simulink model "pgfm_ctrl_analysis"  (R2026b)
settings: Solver=ode23t  StopTime=param.sim.simlength  FixedStep=param.sim.tc  MaxStep=param.glb_time.tc  RelTol=1e-4
values from neighbouring files (symbols this model uses):
  param = add_template_extras(param, options)    [init_model.m]
undefined symbols (not defined in the file or in its folder): magnitude
libraries: fl_lib x99, nesl_utility x59, afe_uvw_ctrl x15, discrete_time_low_pass_filter x3, threephase_inductor_lib x3, dclink_for_two_levels x3, three_phase_pwm_modulator x3, ideal_bridges_lib x3, lithium_ion_battery x1, three_phase_voltage_with_frt_emulator_mfcn x1
(part 4 of 6)

== system pgfm_ctrl_analysis/afe_abc_inv_psm_mod2/AFE_control/afe_control/FRT-VDE4110 ==
  Constant4 : Constant  Value=0
  Mux : Mux
  Mux1 : Mux  Inputs=2
  enable : Step  Time=param.frt.data.settle_time  FinalValue=param.frt.data.enable_frt_1 + param.frt.data.enable_frt_2
  frt_detection_output : Scope  Commented=on  NumInputPorts=3
      settings: ActiveDisplayYMinimum=-0.12499999999999997  ActiveDisplayYMaximum=1.125
  frt_vde4110 : afe_uvw_ctrl/frt_vde4110  p=param.afe.uvw
  positive_reactive_current_reference : Subsystem
  reset : Step  Time=0.025  InitialValue=1  FinalValue=0
  tag scope: frt_active=scoped, i_grid_seq_ref=scoped, pwr_lim_enable=scoped
  wires:
  Mux1/1 -> frt_vde4110/2
  [i_react_pos_ref] -> Mux1/1
  [i_react_neg_ref] -> Mux1/2
  frt_vde4110/1 -> [i_grid_seq_ref]
  Constant4/1 -> [i_react_neg_ref]
  positive_reactive_current_reference/1(i_react_pos_ref) -> [i_react_pos_ref]
  Mux/1 -> frt_vde4110/1
  [v_grid_pos_xi_avg] -> Mux/1
  [v_grid_pos_eta_avg] -> Mux/2
  [v_grid_neg_xi_avg] -> Mux/3
  [v_grid_neg_eta_avg] -> Mux/4
  enable/1 -> frt_vde4110/3  "enable"
  reset/1 -> frt_vde4110/4  "reset"
  frt_vde4110/4 -> frt_detection_output/1  "frt_state"
  frt_vde4110/3 -> frt_detection_output/3, [pwr_lim_enable]  "pwr_lim_enable"
  frt_vde4110/2 -> frt_detection_output/2, [frt_active]  "frt_active"

== system pgfm_ctrl_analysis/afe_abc_inv_psm_mod2/AFE_control/afe_control/current_ctrl ==
  i_xi_ref : Inport
  Mux : Mux  Inputs=3
  current_ctrl_uvw : afe_uvw_ctrl/current_ctrl_uvw  p=param.afe.uvw
  isa_ref/isa : Scope  Commented=on  NumInputPorts=2
      settings: ActiveDisplayYMinimum=-3.5647345146351177  ActiveDisplayYMaximum=2.2290599372806974
  u_alpha_beta_gamma_out : Outport
  wires:
  Mux/1 -> current_ctrl_uvw/2
  current_ctrl_uvw/3 -> isa_ref/isa/2
  current_ctrl_uvw/2 -> isa_ref/isa/1
  current_ctrl_uvw/1 -> u_alpha_beta_gamma_out/1
  [isd_abc_pu] -> current_ctrl_uvw/3
  [phase_grid_pll] -> current_ctrl_uvw/4
  [i_stack_neg_eta_ref] -> Mux/3  "is_neg_eta_ref"
  [i_stack_pos_eta_ref] -> Mux/1  "is_pos_eta_ref"
  [i_stack_neg_xi_ref] -> Mux/2  "is_neg_xi_ref"
  i_xi_ref/1 -> current_ctrl_uvw/1  "is_pos_xi_ref"

== system pgfm_ctrl_analysis/afe_abc_inv_psm_mod2/AFE_control/afe_control/data_to_worspace_module_1 ==
  Bus Creator : BusCreator  Inputs=5
  dq_pll : Subsystem
  inner_current_tracking : Subsystem
  pwr_meter : Subsystem
  sequences_data : Subsystem
  m : Outport
  wires:
  dq_pll/1(dqPLLs) -> Bus Creator/4  "dq_pll"
  [local_time] -> Bus Creator/5  "local_time"
  inner_current_tracking/1(m_inner_current_tracking) -> Bus Creator/3  "m_inner_current_tracking"
  pwr_meter/1(m_pwr_meter) -> Bus Creator/2  "pwr_meter"
  sequences_data/1(m_seq) -> Bus Creator/1  "sequences_data"
  Bus Creator/1 -> m/1

== system pgfm_ctrl_analysis/afe_abc_inv_psm_mod2/AFE_control/afe_control/grid_current_sequences_and_reactive_pwr_ctrl ==
  ig_abc_pu : Inport
  Abs : Abs  SaturateOnIntegerOverflow=off
  Demux : Demux  Outputs=3
  Demux1 : Demux
  Saturation : Saturate  UpperLimit=2  LowerLimit=0.1
  Terminator : Terminator
  grid_current_sequences_q_ctrl : afe_uvw_ctrl/grid_current_sequences_q_ctrl  p=param.afe.uvw
  tag scope: i_grid_neg_eta_avg=scoped, i_grid_neg_xi_avg=scoped, i_grid_pos_eta_avg=scoped, i_grid_pos_xi_avg=scoped, i_stack_neg_eta_ref=scoped, i_stack_neg_xi_ref=scoped, i_stack_pos_eta_ref=scoped
  wires:
  Demux/3 -> [i_stack_neg_eta_ref]
  Demux/2 -> [i_stack_neg_xi_ref]
  Abs/1 -> Saturation/1
  [omega_grid_pll_pu] -> Abs/1
  Saturation/1 -> grid_current_sequences_q_ctrl/3
  [i_grid_seq_ref] -> grid_current_sequences_q_ctrl/4
  grid_current_sequences_q_ctrl/3 -> Terminator/1
  Demux1/4 -> [i_grid_neg_eta_avg]
  Demux1/3 -> [i_grid_neg_xi_avg]
  Demux1/2 -> [i_grid_pos_eta_avg]
  Demux1/1 -> [i_grid_pos_xi_avg]
  grid_current_sequences_q_ctrl/2 -> Demux1/1
  Demux/1 -> [i_stack_pos_eta_ref]
  grid_current_sequences_q_ctrl/1 -> Demux/1
  ig_abc_pu/1 -> grid_current_sequences_q_ctrl/1
  [phase_grid_pll] -> grid_current_sequences_q_ctrl/2

== system pgfm_ctrl_analysis/afe_abc_inv_psm_mod2/AFE_control/afe_control/grid_phase_acquisition ==
  grid_phase : Inport
  Quantizer : Quantizer  QuantizationInterval=param.meas.adc_quantization
  Unit Delay : UnitDelay  SampleTime=-1
  Zero-Order Hold : ZeroOrderHold  SampleTime=-1
  grid_phased : Outport
  wires:
  Quantizer/1 -> Unit Delay/1
  grid_phase/1 -> Zero-Order Hold/1
  Unit Delay/1 -> grid_phased/1
  Zero-Order Hold/1 -> Quantizer/1

== system pgfm_ctrl_analysis/afe_abc_inv_psm_mod2/AFE_control/afe_control/grid_voltage_phase_lock_loops ==
  ug_abc_pu : Inport
  Bus Creator2 : BusCreator  Inputs=2
  FHT-PLL performance : Scope  Commented=on  NumInputPorts=2
      settings: ActiveDisplayYMinimum=-1.32501220703125  ActiveDisplayYMaximum=1.30987548828125  DataLoggingVariableName=ScopeData8
  FHT-PLL_simulink : Subsystem
  tag scope: omega_grid_pll_pu=scoped, phase_grid_pll=scoped
  wires:
  [phase_grid_pll] -> Bus Creator2/1  "phase_grid_fht_pll"
  [omega_grid_pll_pu] -> Bus Creator2/2  "omega_grid_fht_pll"
  Bus Creator2/1 -> FHT-PLL performance/2
  ug_abc_pu/1 -> FHT-PLL_simulink/1(ug_abc_pu), FHT-PLL performance/1
  FHT-PLL_simulink/2(omega_grid_fht_pll) -> [omega_grid_pll_pu]
  FHT-PLL_simulink/1(gamma_grid_fht_pll) -> [phase_grid_pll]

== system pgfm_ctrl_analysis/afe_abc_inv_psm_mod2/AFE_control/afe_control/grid_voltage_sequences ==
  Abs : Abs  SaturateOnIntegerOverflow=off
  Demux : Demux
  Demux1 : Demux  Outputs=2
  Saturation : Saturate  UpperLimit=2  LowerLimit=0.1
  Terminator : Terminator
  grid_voltage_sequences1 : afe_uvw_ctrl/grid_voltage_sequences  p=param.afe.uvw
  tag scope: ug_alpha_pu=scoped, ug_beta_pu=scoped, v_grid_neg_eta_avg=scoped, v_grid_neg_xi_avg=scoped, v_grid_pos_eta_avg=scoped, v_grid_pos_xi_avg=scoped
  wires:
  grid_voltage_sequences1/2 -> Terminator/1
  Demux1/2 -> [ug_beta_pu]
  Demux1/1 -> [ug_alpha_pu]
  grid_voltage_sequences1/3 -> Demux1/1
  Demux/1 -> [v_grid_pos_xi_avg]
  Demux/2 -> [v_grid_pos_eta_avg]
  Demux/3 -> [v_grid_neg_xi_avg]
  Demux/4 -> [v_grid_neg_eta_avg]
  grid_voltage_sequences1/1 -> Demux/1
  Saturation/1 -> grid_voltage_sequences1/3
  [omega_grid_pll_pu] -> Abs/1
  Abs/1 -> Saturation/1
  [phase_grid_pll] -> grid_voltage_sequences1/2
  [ugd_abc_pu] -> grid_voltage_sequences1/1

== system pgfm_ctrl_analysis/afe_abc_inv_psm_mod2/AFE_control/afe_control/i_xi_ref ==
  Constant1 : Constant  Value=param.afe.ref.ixi_ref_mod2
  Constant2 : Constant  Value=0
  Delay : Delay  DelayLength=floor(0.25/param.glb_time.ts_afe)
  Switch : Switch  Criteria=u2 > Threshold  SaturateOnIntegerOverflow=off  InputSameDT=off
  Switch1 : Switch  Criteria=u2 > Threshold  SaturateOnIntegerOverflow=off  InputSameDT=off
  Variant Source : VariantSource  VariantControls={false, true}
  discrete-time-low-pass-filter : discrete_time_low_pass_filter/discrete-time-low-pass-filter  tau=0.125  ts=param.glb_time.ts_afe
  i_xi_ref : Outport
  wires:
  Variant Source/1 -> i_xi_ref/1
  Switch1/1 -> Variant Source/1
  discrete-time-low-pass-filter/1 -> Switch1/1
  Delay/1 -> Switch1/2
  Switch/1 -> Switch1/3, Variant Source/2, discrete-time-low-pass-filter/1
  [pwr_lim_enable] -> Delay/1
  [pwr_lim_enable] -> Switch/2
  Constant2/1 -> Switch/1
  Constant1/1 -> Switch/3  "i_xi_ref"

== system pgfm_ctrl_analysis/afe_abc_inv_psm_mod2/AFE_control/afe_control/ig afe quantizzation and one step delay ==
  ig_abc_pu : Inport
  Demux1 : Demux  Outputs=3
  Mux1 : Mux  Inputs=3
  ig afe quantizzation and one step delay : Subsystem
  igd_abc_pu : Outport
  wires:
  ig afe quantizzation and one step delay/3(igd_w_pu) -> Mux1/3
  ig afe quantizzation and one step delay/1(igd_u_pu) -> Mux1/1
  ig afe quantizzation and one step delay/2(igd_v_pu) -> Mux1/2
  Demux1/3 -> ig afe quantizzation and one step delay/3(ig_w_pu)
  Mux1/1 -> igd_abc_pu/1
  ig_abc_pu/1 -> Demux1/1
  Demux1/2 -> ig afe quantizzation and one step delay/2(ig_v_pu)
  Demux1/1 -> ig afe quantizzation and one step delay/1(ig_u_pu)

== system pgfm_ctrl_analysis/afe_abc_inv_psm_mod2/AFE_control/afe_control/interesting scopes ==
  current_sequences_mod1 : Scope  Commented=on  NumInputPorts=4
      settings: ActiveDisplayYMinimum=-0.97178065031766891  ActiveDisplayYMaximum=1.9392475411295891  DataLoggingVariableName=ScopeData2
  i_grid_seq_ref : Scope  Commented=on
      settings: ActiveDisplayYMinimum=-1.1499999999999995  ActiveDisplayYMaximum=0.34999999999999981
  voltage_sequences_mod1 : Scope  Commented=on  NumInputPorts=4
      settings: ActiveDisplayYMinimum=-1.2405151816982258  ActiveDisplayYMaximum=1.2605257614333911
  wires:
  [i_grid_seq_ref] -> i_grid_seq_ref/1  "i_grid_seq_ref"
  [i_grid_pos_eta_avg] -> current_sequences_mod1/2  "i_grid_pos_eta"
  [v_grid_pos_xi_avg] -> voltage_sequences_mod1/1  "u_grid_pos_xi"
  [i_grid_neg_eta_avg] -> current_sequences_mod1/4  "i_grid_neg_eta"
  [i_grid_pos_xi_avg] -> current_sequences_mod1/1  "i_grid_pos_xi"
  [v_grid_neg_xi_avg] -> voltage_sequences_mod1/3  "u_grid_neg_xi"
  [v_grid_pos_eta_avg] -> voltage_sequences_mod1/2  "u_grid_pos_eta"
  [i_grid_neg_xi_avg] -> current_sequences_mod1/3  "i_grid_neg_xi"
  [v_grid_neg_eta_avg] -> voltage_sequences_mod1/4  "u_grid_neg_eta"

== system pgfm_ctrl_analysis/afe_abc_inv_psm_mod2/AFE_control/afe_control/is afe quantizzation and one step delay ==
  is_abc_pu : Inport
  Demux : Demux  Outputs=3
  Mux : Mux  Inputs=3
  is afe quantizzation and one step delay : Subsystem
  isd_abc_pu : Outport
  wires:
  Demux/2 -> is afe quantizzation and one step delay/2(is_v_pu)
  Demux/3 -> is afe quantizzation and one step delay/3(is_w_pu)
  Mux/1 -> isd_abc_pu/1
  Demux/1 -> is afe quantizzation and one step delay/1(is_u_pu)
  is afe quantizzation and one step delay/1(isd_u_pu) -> Mux/1
  is afe quantizzation and one step delay/3(isd_w_pu) -> Mux/3
  is_abc_pu/1 -> Demux/1
  is afe quantizzation and one step delay/2(isd_v_pu) -> Mux/2

== system pgfm_ctrl_analysis/afe_abc_inv_psm_mod2/AFE_control/afe_control/islanding_mode_detector ==
  gamma : Inport
  alpha : Inport  Port=2
  beta : Inport  Port=3
  Constant : Constant
  Mux : Mux  Inputs=2
  island_detection : Scope  Commented=on  NumInputPorts=3
      settings: ActiveDisplayYMinimum=-13.028939727220205  ActiveDisplayYMaximum=117.26045754498188  DataLoggingVariableName=ScopeData10
  islanding_detector : afe_uvw_ctrl/islanding_detector  p=param.afe.uvw
  wires:
  islanding_detector/3 -> island_detection/3
  islanding_detector/2 -> island_detection/2
  islanding_detector/1 -> island_detection/1
  Constant/1 -> islanding_detector/4
  [omega_grid_pll_pu] -> islanding_detector/3
  gamma/1 -> islanding_detector/2  "gamma_grid"
  beta/1 -> Mux/2  "u_grid_beta"
  alpha/1 -> Mux/1  "u_grid_alpha"
  Mux/1 -> islanding_detector/1

== system pgfm_ctrl_analysis/afe_abc_inv_psm_mod2/AFE_control/afe_control/phase_compensation_1 ==
  local_time : Inport
  master_time : Inport  Port=2
  Zero-Order Hold : ZeroOrderHold  SampleTime=-1
  Zero-Order Hold1 : ZeroOrderHold  SampleTime=-1
  alignment_eval_afe1 : Subsystem
  y : Outport
  wires:
  Zero-Order Hold1/1 -> alignment_eval_afe1/2(master_time)
  Zero-Order Hold/1 -> alignment_eval_afe1/1(local_time)
  alignment_eval_afe1/1(dp) -> y/1
  master_time/1 -> Zero-Order Hold1/1
  local_time/1 -> Zero-Order Hold/1

== system pgfm_ctrl_analysis/afe_abc_inv_psm_mod2/AFE_control/afe_control/space_vector ==
  uab_out : Inport
  Bus Creator : BusCreator  Inputs=3
  Bus Selector : BusSelector  OutputSignals=da,db,dc
  C Caller : CCaller  FunctionName=sv_pwm_cm_process_simulink  PortSpecificationStruct="%)30     .    B H   8    (     @         %    \"     8    !     0         %  0 \"0    $    _    07)G3F%M90  4&]R=$YA;64 4V-O<&4     26YD97@     5'EP90      4VEZ90      27-';&]B86P   X    P    !@    @    $          4    (     0    ,    !         !   P!O=70 #@   #     &    \"     0         !0    @    !     P    $         $  # &]U=  .    .     8    (    !          %    \"     $    &     0         0   ...(+3252 chars)"
  Constant : Constant  Value=param.glb_time.ts_afe
  Constant1 : Constant
  Data Type Conversion1 : DataTypeConversion  OutDataTypeStr=double  SaturateOnIntegerOverflow=off  RndMeth=Floor
  Data Type Conversion{4,15..16,18} (4 alike) : DataTypeConversion  OutDataTypeStr=single  SaturateOnIntegerOverflow=off  RndMeth=Floor
  Data Type Conversion17 : DataTypeConversion  OutDataTypeStr=uint32  SaturateOnIntegerOverflow=off  RndMeth=Floor
  Data Type Conversion2 : DataTypeConversion  OutDataTypeStr=double  SaturateOnIntegerOverflow=off  RndMeth=Floor
  Data Type Conversion3 : DataTypeConversion  OutDataTypeStr=double  SaturateOnIntegerOverflow=off  RndMeth=Floor
  Demux : Demux  Outputs=3
  Gain1 : Gain  Gain=sqrt(3)/2
  Gain2 : Gain  Gain=sqrt(3)/2
  Gain3 : Gain  Gain=param.afe.ref.u_cm_comp_mod2
  duvw : Outport
  wires:
  Data Type Conversion4/1 -> C Caller/3
  Gain3/1 -> Data Type Conversion4/1
  Demux/3 -> Gain3/1
  Data Type Conversion17/1 -> C Caller/5
  Data Type Conversion16/1 -> C Caller/4
  Constant1/1 -> Data Type Conversion17/1
  uab_out/1 -> Demux/1
  Constant/1 -> Data Type Conversion16/1
  Data Type Conversion3/1 -> Bus Creator/3  "dw(k)"
  Gain1/1 -> Data Type Conversion18/1
  Bus Selector/1 -> Data Type Conversion1/1  "<da>"
  Gain2/1 -> Data Type Conversion15/1
  Data Type Conversion2/1 -> Bus Creator/2  "dv(k)"
  Demux/1 -> Gain1/1
  Bus Selector/3 -> Data Type Conversion3/1  "<dc>"
  Demux/2 -> Gain2/1
  Data Type Conversion1/1 -> Bus Creator/1  "du(k)"
  Bus Creator/1 -> duvw/1
  C Caller/1 -> Bus Selector/1
  Data Type Conversion18/1 -> C Caller/1
  Bus Selector/2 -> Data Type Conversion2/1  "<db>"
  Data Type Conversion15/1 -> C Caller/2

== system pgfm_ctrl_analysis/afe_abc_inv_psm_mod2/AFE_control/afe_control/udc_acquisition ==
  udc_pu : Inport
  Quantizer : Quantizer  QuantizationInterval=param.meas.adc_quantization
  Unit Delay : UnitDelay  SampleTime=-1
  Zero-Order Hold : ZeroOrderHold  SampleTime=-1
  udcd_pu : Outport
  wires:
  Zero-Order Hold/1 -> Quantizer/1
  Unit Delay/1 -> udcd_pu/1
  udc_pu/1 -> Zero-Order Hold/1
  Quantizer/1 -> Unit Delay/1

== system pgfm_ctrl_analysis/afe_abc_inv_psm_mod2/AFE_control/afe_control/ug afe quantizzation and one step delay ==
  ug_abc_pu : Inport
  Demux : Demux  Outputs=3
  Mux : Mux  Inputs=3
  ug afe quantizzation and one step delay : Subsystem
  ugd_abc_pu : Outport
  wires:
  Mux/1 -> ugd_abc_pu/1
  ug afe quantizzation and one step delay/3(ugd_w_pu) -> Mux/3
  ug_abc_pu/1 -> Demux/1
  Demux/1 -> ug afe quantizzation and one step delay/1(ug_u_pu)
  ug afe quantizzation and one step delay/1(ugd_u_pu) -> Mux/1
  Demux/3 -> ug afe quantizzation and one step delay/3(ug_w_pu)
  Demux/2 -> ug afe quantizzation and one step delay/2(ug_v_pu)
  ug afe quantizzation and one step delay/2(ugd_v_pu) -> Mux/2

== system pgfm_ctrl_analysis/afe_abc_inv_psm_mod2/afe/sv_pwm/modulator1 ==
  u : Inport
  v : Inport  Port=2
  w : Inport  Port=3
  phase : Inport  Port=4
  Bus Creator : BusCreator  Inputs=3
  Three phase two level PWM generator with global TRGO : three_phase_pwm_modulator/Three phase two level PWM generator with global TRGO  f=param.glb_time.fPWM_AFE  m_up=0.98  m_low=0.02  dead_time=param.glb_time.dead_time_AFE  pos_cmd_gate=15  neg_cmd_gate=-10  polarity=1  tc=param.glb_time.tc  double_sampling=1
      link override gate commands/Bus Selector: OutputSignals=du(t)
      link override gate commands/Bus Selector1: OutputSignals=dv(t)
      link override gate commands/Bus Selector2: OutputSignals=dw(t)
  gate_cmds : Outport
  tag scope: TRGO_afe_module_2=global
  wires:
  Three phase two level PWM generator with global TRGO/2 -> gate_cmds/1
  phase/1 -> Three phase two level PWM generator with global TRGO/2
  w/1 -> Bus Creator/3
  v/1 -> Bus Creator/2
  u/1 -> Bus Creator/1
  Three phase two level PWM generator with global TRGO/1 -> [TRGO_afe_module_2]
  Bus Creator/1 -> Three phase two level PWM generator with global TRGO/3
  [time_afe_module_2] -> Three phase two level PWM generator with global TRGO/1

== system pgfm_ctrl_analysis/afe_abc_inv_psm_mod3/AFE_control/afe_control/FRT-VDE4110 ==
  Constant4 : Constant  Value=0
  Mux : Mux
  Mux1 : Mux  Inputs=2
  enable : Step  Time=param.frt.data.settle_time  FinalValue=param.frt.data.enable_frt_1 + param.frt.data.enable_frt_2
  frt_detection_output : Scope  Commented=on  NumInputPorts=3
      settings: ActiveDisplayYMinimum=-0.12499999999999997  ActiveDisplayYMaximum=1.125
  frt_vde4110 : afe_uvw_ctrl/frt_vde4110  p=param.afe.uvw
  positive_reactive_current_reference : Subsystem
  reset : Step  Time=0.025  InitialValue=1  FinalValue=0
  tag scope: frt_active=scoped, i_grid_seq_ref=scoped, pwr_lim_enable=scoped
  wires:
  frt_vde4110/2 -> [frt_active], frt_detection_output/2  "frt_active"
  frt_vde4110/3 -> [pwr_lim_enable], frt_detection_output/3  "pwr_lim_enable"
  frt_vde4110/4 -> frt_detection_output/1  "frt_state"
  reset/1 -> frt_vde4110/4  "reset"
  enable/1 -> frt_vde4110/3  "enable"
  [v_grid_neg_eta_avg] -> Mux/4
  [v_grid_neg_xi_avg] -> Mux/3
  [v_grid_pos_eta_avg] -> Mux/2
  [v_grid_pos_xi_avg] -> Mux/1
  Mux/1 -> frt_vde4110/1
  positive_reactive_current_reference/1(i_react_pos_ref) -> [i_react_pos_ref]
  Constant4/1 -> [i_react_neg_ref]
  frt_vde4110/1 -> [i_grid_seq_ref]
  [i_react_neg_ref] -> Mux1/2
  [i_react_pos_ref] -> Mux1/1
  Mux1/1 -> frt_vde4110/2

== system pgfm_ctrl_analysis/afe_abc_inv_psm_mod3/AFE_control/afe_control/current_ctrl ==
  i_xi_ref : Inport
  Mux : Mux  Inputs=3
  current_ctrl_uvw : afe_uvw_ctrl/current_ctrl_uvw  p=param.afe.uvw
  isa_ref/isa : Scope  Commented=on  NumInputPorts=2
      settings: ActiveDisplayYMinimum=-3.5647345146351177  ActiveDisplayYMaximum=2.2290599372806974
  u_alpha_beta_gamma_out : Outport
  wires:
  i_xi_ref/1 -> current_ctrl_uvw/1  "is_pos_xi_ref"
  [i_stack_neg_xi_ref] -> Mux/2  "is_neg_xi_ref"
  [i_stack_pos_eta_ref] -> Mux/1  "is_pos_eta_ref"
  [i_stack_neg_eta_ref] -> Mux/3  "is_neg_eta_ref"
  [phase_grid_pll] -> current_ctrl_uvw/4
  [isd_abc_pu] -> current_ctrl_uvw/3
  current_ctrl_uvw/1 -> u_alpha_beta_gamma_out/1
  current_ctrl_uvw/2 -> isa_ref/isa/1
  current_ctrl_uvw/3 -> isa_ref/isa/2
  Mux/1 -> current_ctrl_uvw/2

== system pgfm_ctrl_analysis/afe_abc_inv_psm_mod3/AFE_control/afe_control/data_to_worspace_module_1 ==
  Bus Creator : BusCreator  Inputs=5
  dq_pll : Subsystem
  inner_current_tracking : Subsystem
  pwr_meter : Subsystem
  sequences_data : Subsystem
  m : Outport
  wires:
  Bus Creator/1 -> m/1
  sequences_data/1(m_seq) -> Bus Creator/1  "sequences_data"
  pwr_meter/1(m_pwr_meter) -> Bus Creator/2  "pwr_meter"
  inner_current_tracking/1(m_inner_current_tracking) -> Bus Creator/3  "m_inner_current_tracking"
  [local_time] -> Bus Creator/5  "local_time"
  dq_pll/1(dqPLLs) -> Bus Creator/4  "dq_pll"

== system pgfm_ctrl_analysis/afe_abc_inv_psm_mod3/AFE_control/afe_control/grid_current_sequences_and_reactive_pwr_ctrl ==
  ig_abc_pu : Inport
  Abs : Abs  SaturateOnIntegerOverflow=off
  Demux : Demux  Outputs=3
  Demux1 : Demux
  Saturation : Saturate  UpperLimit=2  LowerLimit=0.1
  Terminator : Terminator
  grid_current_sequences_q_ctrl : afe_uvw_ctrl/grid_current_sequences_q_ctrl  p=param.afe.uvw
  tag scope: i_grid_neg_eta_avg=scoped, i_grid_neg_xi_avg=scoped, i_grid_pos_eta_avg=scoped, i_grid_pos_xi_avg=scoped, i_stack_neg_eta_ref=scoped, i_stack_neg_xi_ref=scoped, i_stack_pos_eta_ref=scoped
  wires:
  [phase_grid_pll] -> grid_current_sequences_q_ctrl/2
  ig_abc_pu/1 -> grid_current_sequences_q_ctrl/1
  grid_current_sequences_q_ctrl/1 -> Demux/1
  Demux/1 -> [i_stack_pos_eta_ref]
  grid_current_sequences_q_ctrl/2 -> Demux1/1
  Demux1/1 -> [i_grid_pos_xi_avg]
  Demux1/2 -> [i_grid_pos_eta_avg]
  Demux1/3 -> [i_grid_neg_xi_avg]
  Demux1/4 -> [i_grid_neg_eta_avg]
  grid_current_sequences_q_ctrl/3 -> Terminator/1
  [i_grid_seq_ref] -> grid_current_sequences_q_ctrl/4
  Saturation/1 -> grid_current_sequences_q_ctrl/3
  [omega_grid_pll_pu] -> Abs/1
  Abs/1 -> Saturation/1
  Demux/2 -> [i_stack_neg_xi_ref]
  Demux/3 -> [i_stack_neg_eta_ref]

== system pgfm_ctrl_analysis/afe_abc_inv_psm_mod3/AFE_control/afe_control/grid_phase_acquisition ==
  grid_phase : Inport
  Quantizer : Quantizer  QuantizationInterval=param.meas.adc_quantization
  Unit Delay : UnitDelay  SampleTime=-1
  Zero-Order Hold : ZeroOrderHold  SampleTime=-1
  grid_phased : Outport
  wires:
  Zero-Order Hold/1 -> Quantizer/1
  Unit Delay/1 -> grid_phased/1
  grid_phase/1 -> Zero-Order Hold/1
  Quantizer/1 -> Unit Delay/1

== system pgfm_ctrl_analysis/afe_abc_inv_psm_mod3/AFE_control/afe_control/grid_voltage_phase_lock_loops ==
  ug_abc_pu : Inport
  Bus Creator2 : BusCreator  Inputs=2
  FHT-PLL performance : Scope  Commented=on  NumInputPorts=2
      settings: ActiveDisplayYMinimum=-1.32501220703125  ActiveDisplayYMaximum=1.30987548828125  DataLoggingVariableName=ScopeData8
  FHT-PLL_simulink : Subsystem
  tag scope: omega_grid_pll_pu=scoped, phase_grid_pll=scoped
  wires:
  FHT-PLL_simulink/1(gamma_grid_fht_pll) -> [phase_grid_pll]
  FHT-PLL_simulink/2(omega_grid_fht_pll) -> [omega_grid_pll_pu]
  ug_abc_pu/1 -> FHT-PLL performance/1, FHT-PLL_simulink/1(ug_abc_pu)
  Bus Creator2/1 -> FHT-PLL performance/2
  [omega_grid_pll_pu] -> Bus Creator2/2  "omega_grid_fht_pll"
  [phase_grid_pll] -> Bus Creator2/1  "phase_grid_fht_pll"

== system pgfm_ctrl_analysis/afe_abc_inv_psm_mod3/AFE_control/afe_control/grid_voltage_sequences ==
  Abs : Abs  SaturateOnIntegerOverflow=off
  Demux : Demux
  Demux1 : Demux  Outputs=2
  Saturation : Saturate  UpperLimit=2  LowerLimit=0.1
  Terminator : Terminator
  grid_voltage_sequences1 : afe_uvw_ctrl/grid_voltage_sequences  p=param.afe.uvw
  tag scope: ug_alpha_pu=scoped, ug_beta_pu=scoped, v_grid_neg_eta_avg=scoped, v_grid_neg_xi_avg=scoped, v_grid_pos_eta_avg=scoped, v_grid_pos_xi_avg=scoped
  wires:
  [ugd_abc_pu] -> grid_voltage_sequences1/1
  [phase_grid_pll] -> grid_voltage_sequences1/2
  Abs/1 -> Saturation/1
  [omega_grid_pll_pu] -> Abs/1
  Saturation/1 -> grid_voltage_sequences1/3
  grid_voltage_sequences1/1 -> Demux/1
  Demux/4 -> [v_grid_neg_eta_avg]
  Demux/3 -> [v_grid_neg_xi_avg]
  Demux/2 -> [v_grid_pos_eta_avg]
  Demux/1 -> [v_grid_pos_xi_avg]
  grid_voltage_sequences1/3 -> Demux1/1
  Demux1/1 -> [ug_alpha_pu]
  Demux1/2 -> [ug_beta_pu]
  grid_voltage_sequences1/2 -> Terminator/1

== system pgfm_ctrl_analysis/afe_abc_inv_psm_mod3/AFE_control/afe_control/i_xi_ref ==
  Constant1 : Constant  Value=param.afe.ref.ixi_ref_mod3
  Constant2 : Constant  Value=0
  Delay : Delay  DelayLength=floor(0.25/param.glb_time.ts_afe)
  Switch : Switch  Criteria=u2 > Threshold  SaturateOnIntegerOverflow=off  InputSameDT=off
  Switch1 : Switch  Criteria=u2 > Threshold  SaturateOnIntegerOverflow=off  InputSameDT=off
  Variant Source : VariantSource  VariantControls={false, true}
  discrete-time-low-pass-filter : discrete_time_low_pass_filter/discrete-time-low-pass-filter  tau=0.125  ts=param.glb_time.ts_afe
  i_xi_ref : Outport
  wires:
  Constant1/1 -> Switch/3  "i_xi_ref"
  Constant2/1 -> Switch/1
  [pwr_lim_enable] -> Switch/2
  [pwr_lim_enable] -> Delay/1
  Switch/1 -> discrete-time-low-pass-filter/1, Variant Source/2, Switch1/3
  Delay/1 -> Switch1/2
  discrete-time-low-pass-filter/1 -> Switch1/1
  Switch1/1 -> Variant Source/1
  Variant Source/1 -> i_xi_ref/1

== system pgfm_ctrl_analysis/afe_abc_inv_psm_mod3/AFE_control/afe_control/ig afe quantizzation and one step delay ==
  ig_abc_pu : Inport
  Demux1 : Demux  Outputs=3
  Mux1 : Mux  Inputs=3
  ig afe quantizzation and one step delay : Subsystem
  igd_abc_pu : Outport
  wires:
  Demux1/1 -> ig afe quantizzation and one step delay/1(ig_u_pu)
  Demux1/2 -> ig afe quantizzation and one step delay/2(ig_v_pu)
  ig_abc_pu/1 -> Demux1/1
  Mux1/1 -> igd_abc_pu/1
  Demux1/3 -> ig afe quantizzation and one step delay/3(ig_w_pu)
  ig afe quantizzation and one step delay/2(igd_v_pu) -> Mux1/2
  ig afe quantizzation and one step delay/1(igd_u_pu) -> Mux1/1
  ig afe quantizzation and one step delay/3(igd_w_pu) -> Mux1/3

== system pgfm_ctrl_analysis/afe_abc_inv_psm_mod3/AFE_control/afe_control/interesting scopes ==
  current_sequences_mod1 : Scope  Commented=on  NumInputPorts=4
      settings: ActiveDisplayYMinimum=-0.97178065031766891  ActiveDisplayYMaximum=1.9392475411295891  DataLoggingVariableName=ScopeData2
  i_grid_seq_ref : Scope  Commented=on
      settings: ActiveDisplayYMinimum=-1.1499999999999995  ActiveDisplayYMaximum=0.34999999999999981
  voltage_sequences_mod1 : Scope  Commented=on  NumInputPorts=4
      settings: ActiveDisplayYMinimum=-1.2405151816982258  ActiveDisplayYMaximum=1.2605257614333911
  wires:
  [v_grid_neg_eta_avg] -> voltage_sequences_mod1/4  "u_grid_neg_eta"
  [i_grid_neg_xi_avg] -> current_sequences_mod1/3  "i_grid_neg_xi"
  [v_grid_pos_eta_avg] -> voltage_sequences_mod1/2  "u_grid_pos_eta"
  [v_grid_neg_xi_avg] -> voltage_sequences_mod1/3  "u_grid_neg_xi"
  [i_grid_pos_xi_avg] -> current_sequences_mod1/1  "i_grid_pos_xi"
  [i_grid_neg_eta_avg] -> current_sequences_mod1/4  "i_grid_neg_eta"
  [v_grid_pos_xi_avg] -> voltage_sequences_mod1/1  "u_grid_pos_xi"
  [i_grid_pos_eta_avg] -> current_sequences_mod1/2  "i_grid_pos_eta"
  [i_grid_seq_ref] -> i_grid_seq_ref/1  "i_grid_seq_ref"

== system pgfm_ctrl_analysis/afe_abc_inv_psm_mod3/AFE_control/afe_control/is afe quantizzation and one step delay ==
  is_abc_pu : Inport
  Demux : Demux  Outputs=3
  Mux : Mux  Inputs=3
  is afe quantizzation and one step delay : Subsystem
  isd_abc_pu : Outport
  wires:
  is afe quantizzation and one step delay/2(isd_v_pu) -> Mux/2
  is_abc_pu/1 -> Demux/1
  is afe quantizzation and one step delay/3(isd_w_pu) -> Mux/3
  is afe quantizzation and one step delay/1(isd_u_pu) -> Mux/1
  Demux/1 -> is afe quantizzation and one step delay/1(is_u_pu)
  Mux/1 -> isd_abc_pu/1
  Demux/3 -> is afe quantizzation and one step delay/3(is_w_pu)
  Demux/2 -> is afe quantizzation and one step delay/2(is_v_pu)

== system pgfm_ctrl_analysis/afe_abc_inv_psm_mod3/AFE_control/afe_control/islanding_mode_detector ==
  gamma : Inport
  alpha : Inport  Port=2
  beta : Inport  Port=3
  Constant : Constant
  Mux : Mux  Inputs=2
  island_detection : Scope  Commented=on  NumInputPorts=3
      settings: ActiveDisplayYMinimum=-13.028939727220205  ActiveDisplayYMaximum=117.26045754498188  DataLoggingVariableName=ScopeData10
  islanding_detector : afe_uvw_ctrl/islanding_detector  p=param.afe.uvw
  wires:
  Mux/1 -> islanding_detector/1
  alpha/1 -> Mux/1  "u_grid_alpha"
  beta/1 -> Mux/2  "u_grid_beta"
  gamma/1 -> islanding_detector/2  "gamma_grid"
  [omega_grid_pll_pu] -> islanding_detector/3
  Constant/1 -> islanding_detector/4
  islanding_detector/1 -> island_detection/1
  islanding_detector/2 -> island_detection/2
  islanding_detector/3 -> island_detection/3

== system pgfm_ctrl_analysis/afe_abc_inv_psm_mod3/AFE_control/afe_control/phase_compensation_1 ==
  local_time : Inport
  master_time : Inport  Port=2
  Zero-Order Hold : ZeroOrderHold  SampleTime=-1
  Zero-Order Hold1 : ZeroOrderHold  SampleTime=-1
  alignment_eval_afe1 : Subsystem
  y : Outport
  wires:
  local_time/1 -> Zero-Order Hold/1
  master_time/1 -> Zero-Order Hold1/1
  alignment_eval_afe1/1(dp) -> y/1
  Zero-Order Hold/1 -> alignment_eval_afe1/1(local_time)
  Zero-Order Hold1/1 -> alignment_eval_afe1/2(master_time)

== system pgfm_ctrl_analysis/afe_abc_inv_psm_mod3/AFE_control/afe_control/space_vector ==
  uab_out : Inport
  Bus Creator : BusCreator  Inputs=3
  Bus Selector : BusSelector  OutputSignals=da,db,dc
  C Caller : CCaller  FunctionName=sv_pwm_cm_process_simulink  PortSpecificationStruct="%)30     .    B H   8    (     @         %    \"     8    !     0         %  0 \"0    $    _    07)G3F%M90  4&]R=$YA;64 4V-O<&4     26YD97@     5'EP90      4VEZ90      27-';&]B86P   X    P    !@    @    $          4    (     0    ,    !         !   P!O=70 #@   #     &    \"     0         !0    @    !     P    $         $  # &]U=  .    .     8    (    !          %    \"     $    &     0         0   ...(+3252 chars)"
  Constant : Constant  Value=param.glb_time.ts_afe
  Constant1 : Constant
  Data Type Conversion1 : DataTypeConversion  OutDataTypeStr=double  SaturateOnIntegerOverflow=off  RndMeth=Floor
  Data Type Conversion{4,15..16,18} (4 alike) : DataTypeConversion  OutDataTypeStr=single  SaturateOnIntegerOverflow=off  RndMeth=Floor
  Data Type Conversion17 : DataTypeConversion  OutDataTypeStr=uint32  SaturateOnIntegerOverflow=off  RndMeth=Floor
  Data Type Conversion2 : DataTypeConversion  OutDataTypeStr=double  SaturateOnIntegerOverflow=off  RndMeth=Floor
  Data Type Conversion3 : DataTypeConversion  OutDataTypeStr=double  SaturateOnIntegerOverflow=off  RndMeth=Floor
  Demux : Demux  Outputs=3
  Gain1 : Gain  Gain=sqrt(3)/2
  Gain2 : Gain  Gain=sqrt(3)/2
  Gain3 : Gain  Gain=param.afe.ref.u_cm_comp_mod3
  duvw : Outport
  wires:
  Data Type Conversion15/1 -> C Caller/2
  Bus Selector/2 -> Data Type Conversion2/1  "<db>"
  Data Type Conversion18/1 -> C Caller/1
  C Caller/1 -> Bus Selector/1
  Bus Creator/1 -> duvw/1
  Data Type Conversion1/1 -> Bus Creator/1  "du(k)"
  Demux/2 -> Gain2/1
  Bus Selector/3 -> Data Type Conversion3/1  "<dc>"
  Demux/1 -> Gain1/1
  Data Type Conversion2/1 -> Bus Creator/2  "dv(k)"
  Gain2/1 -> Data Type Conversion15/1
  Bus Selector/1 -> Data Type Conversion1/1  "<da>"
  Gain1/1 -> Data Type Conversion18/1
  Data Type Conversion3/1 -> Bus Creator/3  "dw(k)"
  Constant/1 -> Data Type Conversion16/1
  uab_out/1 -> Demux/1
  Constant1/1 -> Data Type Conversion17/1
  Data Type Conversion16/1 -> C Caller/4
  Data Type Conversion17/1 -> C Caller/5
  Demux/3 -> Gain3/1
  Gain3/1 -> Data Type Conversion4/1
  Data Type Conversion4/1 -> C Caller/3

== system pgfm_ctrl_analysis/afe_abc_inv_psm_mod3/AFE_control/afe_control/udc_acquisition ==
  udc_pu : Inport
  Quantizer : Quantizer  QuantizationInterval=param.meas.adc_quantization
  Unit Delay : UnitDelay  SampleTime=-1
  Zero-Order Hold : ZeroOrderHold  SampleTime=-1
  udcd_pu : Outport
  wires:
  Quantizer/1 -> Unit Delay/1
  udc_pu/1 -> Zero-Order Hold/1
  Unit Delay/1 -> udcd_pu/1
  Zero-Order Hold/1 -> Quantizer/1

== system pgfm_ctrl_analysis/afe_abc_inv_psm_mod3/AFE_control/afe_control/ug afe quantizzation and one step delay ==
  ug_abc_pu : Inport
  Demux : Demux  Outputs=3
  Mux : Mux  Inputs=3
  ug afe quantizzation and one step delay : Subsystem
  ugd_abc_pu : Outport
  wires:
  ug afe quantizzation and one step delay/2(ugd_v_pu) -> Mux/2
  Demux/2 -> ug afe quantizzation and one step delay/2(ug_v_pu)
  Demux/3 -> ug afe quantizzation and one step delay/3(ug_w_pu)
  ug afe quantizzation and one step delay/1(ugd_u_pu) -> Mux/1
  Demux/1 -> ug afe quantizzation and one step delay/1(ug_u_pu)
  ug_abc_pu/1 -> Demux/1
  ug afe quantizzation and one step delay/3(ugd_w_pu) -> Mux/3
  Mux/1 -> ugd_abc_pu/1

== system pgfm_ctrl_analysis/afe_abc_inv_psm_mod3/afe/sv_pwm/modulator1 ==
  u : Inport
  v : Inport  Port=2
  w : Inport  Port=3
  phase : Inport  Port=4
  Bus Creator : BusCreator  Inputs=3
  Three phase two level PWM generator with global TRGO : three_phase_pwm_modulator/Three phase two level PWM generator with global TRGO  f=param.glb_time.fPWM_AFE  m_up=0.98  m_low=0.02  dead_time=param.glb_time.dead_time_AFE  pos_cmd_gate=15  neg_cmd_gate=-10  polarity=1  tc=param.glb_time.tc  double_sampling=1
      link override gate commands/Bus Selector: OutputSignals=du(t)
      link override gate commands/Bus Selector1: OutputSignals=dv(t)
      link override gate commands/Bus Selector2: OutputSignals=dw(t)
  gate_cmds : Outport
  tag scope: TRGO_afe_module_3=global
  wires:
  [time_afe_module_3] -> Three phase two level PWM generator with global TRGO/1
  Bus Creator/1 -> Three phase two level PWM generator with global TRGO/3
  Three phase two level PWM generator with global TRGO/1 -> [TRGO_afe_module_3]
  u/1 -> Bus Creator/1
  v/1 -> Bus Creator/2
  w/1 -> Bus Creator/3
  phase/1 -> Three phase two level PWM generator with global TRGO/2
  Three phase two level PWM generator with global TRGO/2 -> gate_cmds/1

== system pgfm_ctrl_analysis/afe_abc_inv_psm_mod1/AFE_control/afe_control/FRT-VDE4110/positive_reactive_current_reference ==
  Step : Step  Time=param.afe.ref.time_i_react_pos_ref_1  InitialValue=param.afe.ref.i_react_pos_ref_1  FinalValue=param.afe.ref.i_react_pos_ref_2
  Step1 : Step  Time=param.afe.ref.time_i_react_pos_ref_2  FinalValue=param.afe.ref.i_react_pos_ref_3-param.afe.ref.i_react_pos_ref_2
  Sum7 : Sum  Inputs=|++
  i_react_pos_ref : Outport
  wires:
  Sum7/1 -> i_react_pos_ref/1
  Step1/1 -> Sum7/2
  Step/1 -> Sum7/1

== system pgfm_ctrl_analysis/afe_abc_inv_psm_mod1/AFE_control/afe_control/data_to_worspace_module_1/dq_pll ==
  Bus Creator1 : BusCreator  Inputs=8
  dqPLLs : Outport
  wires:
  [phase_grid_fht_simulink_pll] -> Bus Creator1/5  "phase_grid_fht_simulink_pll"
  [omega_grid_fht_simulink_pll] -> Bus Creator1/6  "omega_grid_fht_simulink_pll"
  [omega_grid_fhtsr_dqpll] -> Bus Creator1/8  "omega_grid_fhtsr_dqpll"
  [phase_grid_fhtsr_dqpll] -> Bus Creator1/7  "phase_grid_fhtsr_dqpll"
  [omega_grid_dqpll_ccaller] -> Bus Creator1/4  "omega_grid_dqpll_ccaller"
  [phase_grid_dqpll_ccaller] -> Bus Creator1/3  "phase_grid_dqpll_ccaller"
  [omega_grid_pu_dqpll] -> Bus Creator1/2  "omega_grid_pu_dqpll"
  [phase_grid_dqpll] -> Bus Creator1/1  "phase_grid_dqpll"
  Bus Creator1/1 -> dqPLLs/1

== system pgfm_ctrl_analysis/afe_abc_inv_psm_mod1/AFE_control/afe_control/data_to_worspace_module_1/inner_current_tracking ==
  Bus Creator1 : BusCreator  Inputs=11
  m_inner_current_tracking : Outport
  wires:
  [iz_pu] -> Bus Creator1/10  "iz_pu"
  [id_eta_pu] -> Bus Creator1/2  "i_eta_pu"
  [isc] -> Bus Creator1/8  "isc_pu"
  [isa_ref] -> Bus Creator1/3  "isa_pu_ref"
  [isa] -> Bus Creator1/4  "isa_pu"
  [id_xi_pu] -> Bus Creator1/1  "i_xi_pu"
  [iz_pu_ref] -> Bus Creator1/9  "iz_pu_ref"
  [isb] -> Bus Creator1/6  "isb_pu"
  [isb_ref] -> Bus Creator1/5  "isb_pu_ref"
  [iz_ctrl_out] -> Bus Creator1/11  "iz_ctrl_out"
  [isc_ref] -> Bus Creator1/7  "isc_pu_ref"
  Bus Creator1/1 -> m_inner_current_tracking/1

== system pgfm_ctrl_analysis/afe_abc_inv_psm_mod1/AFE_control/afe_control/data_to_worspace_module_1/pwr_meter ==
  Bus Creator1 : BusCreator  Inputs=4
  m_pwr_meter : Outport
  wires:
  [u_grid_pu_rms] -> Bus Creator1/2  "u_grid_pu_rms"
  Bus Creator1/1 -> m_pwr_meter/1
  [pwr_act_grid] -> Bus Creator1/3  "pwr_act_grid"
  [pwr_react_grid] -> Bus Creator1/4  "pwr_react_grid"
  [i_grid_pu_rms] -> Bus Creator1/1  "i_grid_pu_rms"

== system pgfm_ctrl_analysis/afe_abc_inv_psm_mod1/AFE_control/afe_control/data_to_worspace_module_1/sequences_data ==
  Bus Creator1 : BusCreator  Inputs=11
  Demux : Demux  Outputs=3
  m_seq : Outport
  wires:
  Bus Creator1/1 -> m_seq/1
  Demux/3 -> Bus Creator1/3  "i_grid_neg_eta_ref"
  Demux/2 -> Bus Creator1/2  "i_grid_neg_xi_ref"
  Demux/1 -> Bus Creator1/1  "i_grid_pos_eta_ref"
  [v_grid_pos_xi_avg] -> Bus Creator1/4  "v_grid_pos_xi_avg"
  [v_grid_pos_eta_avg] -> Bus Creator1/5  "v_grid_pos_eta_avg"
  [v_grid_neg_xi_avg] -> Bus Creator1/6  "v_grid_neg_xi_avg"
  [v_grid_neg_eta_avg] -> Bus Creator1/7  "v_grid_neg_eta_avg"
  [i_grid_pos_xi_avg] -> Bus Creator1/8  "i_grid_pos_xi_avg"
  [i_grid_pos_eta_avg] -> Bus Creator1/9  "i_grid_pos_eta_avg"
  [i_grid_neg_xi_avg] -> Bus Creator1/10  "i_grid_neg_xi_avg"
  [i_grid_neg_eta_avg] -> Bus Creator1/11  "i_grid_neg_eta_avg"
  [i_grid_seq_ref] -> Demux/1

== system pgfm_ctrl_analysis/afe_abc_inv_psm_mod1/AFE_control/afe_control/grid_voltage_phase_lock_loops/FHT-PLL_simulink ==
  ug_abc_pu : Inport
  pll_stageA : Subsystem
  pll_stageB : Subsystem
  gamma_grid_fht_pll : Outport
  omega_grid_fht_pll : Outport  Port=2
  wires:
  pll_stageB/1(gamma_grid_ddsrf_pll) -> pll_stageA/1(gamma_grid), gamma_grid_fht_pll/1
  pll_stageA/2(u_grid_eta) -> pll_stageB/2(u_grid_pos_eta)  "u_grid_pos_eta"
  pll_stageA/1(u_grid_xi) -> pll_stageB/1(u_grid_pos_xi)  "u_grid_pos_xi"
  pll_stageB/2(omega_grid_ddsrf_pll) -> omega_grid_fht_pll/1
  ug_abc_pu/1 -> pll_stageA/2(ug_abc_pu)

== system pgfm_ctrl_analysis/afe_abc_inv_psm_mod1/AFE_control/afe_control/ig afe quantizzation and one step delay/ig afe quantizzation and one step delay ==
  ig_u_pu : Inport
  ig_v_pu : Inport  Port=2
  ig_w_pu : Inport  Port=3
  Gain4 : Gain  Gain=-1
  Gain5 : Gain  Gain=-1
  Gain6 : Gain  Gain=-1
  Quantizer1 : Quantizer  QuantizationInterval=param.meas.adc_quantization
  Quantizer2 : Quantizer  QuantizationInterval=param.meas.adc_quantization
  Quantizer4 : Quantizer  QuantizationInterval=param.meas.adc_quantization
  Unit Delay : UnitDelay  SampleTime=-1
  Unit Delay1 : UnitDelay  SampleTime=-1
  Unit Delay2 : UnitDelay  SampleTime=-1
  Zero-Order Hold : ZeroOrderHold  SampleTime=-1
  Zero-Order Hold1 : ZeroOrderHold  SampleTime=-1
  Zero-Order Hold2 : ZeroOrderHold  SampleTime=-1
  igd_u_pu : Outport
  igd_v_pu : Outport  Port=2
  igd_w_pu : Outport  Port=3
  wires:
  Quantizer1/1 -> Unit Delay1/1
  Quantizer4/1 -> Unit Delay/1
  Quantizer2/1 -> Unit Delay2/1
  ig_u_pu/1 -> Zero-Order Hold/1
  ig_v_pu/1 -> Zero-Order Hold1/1
  ig_w_pu/1 -> Zero-Order Hold2/1
  Unit Delay/1 -> Gain4/1
  Unit Delay1/1 -> Gain5/1
  Unit Delay2/1 -> Gain6/1
  Gain4/1 -> igd_u_pu/1
  Gain5/1 -> igd_v_pu/1
  Gain6/1 -> igd_w_pu/1
  Zero-Order Hold/1 -> Quantizer4/1
  Zero-Order Hold1/1 -> Quantizer1/1
  Zero-Order Hold2/1 -> Quantizer2/1

== system pgfm_ctrl_analysis/afe_abc_inv_psm_mod1/AFE_control/afe_control/is afe quantizzation and one step delay/is afe quantizzation and one step delay ==
  is_u_pu : Inport
  is_v_pu : Inport  Port=2
  is_w_pu : Inport  Port=3
  Quantizer : Quantizer  QuantizationInterval=param.meas.adc_quantization
  Quantizer1 : Quantizer  QuantizationInterval=param.meas.adc_quantization
  Quantizer2 : Quantizer  QuantizationInterval=param.meas.adc_quantization
  Unit Delay : UnitDelay  SampleTime=-1
  Unit Delay1 : UnitDelay  SampleTime=-1
  Unit Delay2 : UnitDelay  SampleTime=-1
  Zero-Order Hold : ZeroOrderHold  SampleTime=-1
  Zero-Order Hold1 : ZeroOrderHold  SampleTime=-1
  Zero-Order Hold2 : ZeroOrderHold  SampleTime=-1
  isd_u_pu : Outport
  isd_v_pu : Outport  Port=2
  isd_w_pu : Outport  Port=3
  wires:
  Unit Delay/1 -> isd_u_pu/1
  Unit Delay1/1 -> isd_v_pu/1
  Unit Delay2/1 -> isd_w_pu/1
  Quantizer/1 -> Unit Delay/1
  Quantizer1/1 -> Unit Delay1/1
  Quantizer2/1 -> Unit Delay2/1
  is_u_pu/1 -> Zero-Order Hold/1
  is_v_pu/1 -> Zero-Order Hold1/1
  is_w_pu/1 -> Zero-Order Hold2/1
  Zero-Order Hold/1 -> Quantizer/1
  Zero-Order Hold1/1 -> Quantizer1/1
  Zero-Order Hold2/1 -> Quantizer2/1

== system pgfm_ctrl_analysis/afe_abc_inv_psm_mod1/AFE_control/afe_control/phase_compensation_1/alignment_eval_afe1 ==
  local_time : Inport
  master_time : Inport  Port=2
  Constant : Constant  Value=0
  Gain : Gain  Gain=-1
  Sum : Sum  Inputs=|+-
  pi : Subsystem  mask{kp=param.ctrl.kp_align, ki=param.ctrl.ki_align*param.glb_time.ts_afe, lim_up=param.ctrl.lim_up_align, lim_down=param.ctrl.lim_down_align}
      mask prompts: ki "ki*ts"
      mask Display:
      | disp('pi()');
      | port_label('input', 1, 'u_ref');
      | port_label('input', 2, 'u');
      | port_label('output', 1, 'y');
  dp : Outport
  wires:
  master_time/1 -> Sum/1
  Sum/1 -> Gain/1
  Constant/1 -> pi/1(u_ref)
  local_time/1 -> Sum/2
  Gain/1 -> pi/2(u)
  pi/1(y) -> dp/1

== system pgfm_ctrl_analysis/afe_abc_inv_psm_mod1/AFE_control/afe_control/ug afe quantizzation and one step delay/ug afe quantizzation and one step delay ==
  ug_u_pu : Inport
  ug_v_pu : Inport  Port=2
  ug_w_pu : Inport  Port=3
  Quantizer1 : Quantizer  QuantizationInterval=param.meas.adc_quantization
  Quantizer2 : Quantizer  QuantizationInterval=param.meas.adc_quantization
  Quantizer4 : Quantizer  QuantizationInterval=param.meas.adc_quantization
  Unit Delay : UnitDelay  SampleTime=-1
  Unit Delay1 : UnitDelay  SampleTime=-1
  Unit Delay2 : UnitDelay  SampleTime=-1
  Zero-Order Hold : ZeroOrderHold  SampleTime=-1
  Zero-Order Hold1 : ZeroOrderHold  SampleTime=-1
  Zero-Order Hold2 : ZeroOrderHold  SampleTime=-1
  ugd_u_pu : Outport
  ugd_v_pu : Outport  Port=2
  ugd_w_pu : Outport  Port=3
  wires:
  Unit Delay/1 -> ugd_u_pu/1
  Unit Delay1/1 -> ugd_v_pu/1
  Unit Delay2/1 -> ugd_w_pu/1
  Quantizer4/1 -> Unit Delay/1
  Quantizer1/1 -> Unit Delay1/1
  Quantizer2/1 -> Unit Delay2/1
  ug_w_pu/1 -> Zero-Order Hold2/1
  ug_v_pu/1 -> Zero-Order Hold1/1
  ug_u_pu/1 -> Zero-Order Hold/1
  Zero-Order Hold/1 -> Quantizer4/1
  Zero-Order Hold1/1 -> Quantizer1/1
  Zero-Order Hold2/1 -> Quantizer2/1

== system pgfm_ctrl_analysis/afe_abc_inv_psm_mod2/AFE_control/afe_control/FRT-VDE4110/positive_reactive_current_reference ==
  Step : Step  Time=param.afe.ref.time_i_react_pos_ref_1  InitialValue=param.afe.ref.i_react_pos_ref_1  FinalValue=param.afe.ref.i_react_pos_ref_2
  Step1 : Step  Time=param.afe.ref.time_i_react_pos_ref_2  FinalValue=param.afe.ref.i_react_pos_ref_3-param.afe.ref.i_react_pos_ref_2
  Sum7 : Sum  Inputs=|++
  i_react_pos_ref : Outport
  wires:
  Step/1 -> Sum7/1
  Step1/1 -> Sum7/2
  Sum7/1 -> i_react_pos_ref/1

== system pgfm_ctrl_analysis/afe_abc_inv_psm_mod2/AFE_control/afe_control/data_to_worspace_module_1/dq_pll ==
  Bus Creator1 : BusCreator  Inputs=8
  dqPLLs : Outport
  wires:
  Bus Creator1/1 -> dqPLLs/1
  [phase_grid_dqpll] -> Bus Creator1/1  "phase_grid_dqpll"
  [omega_grid_pu_dqpll] -> Bus Creator1/2  "omega_grid_pu_dqpll"
  [phase_grid_dqpll_ccaller] -> Bus Creator1/3  "phase_grid_dqpll_ccaller"
  [omega_grid_dqpll_ccaller] -> Bus Creator1/4  "omega_grid_dqpll_ccaller"
  [phase_grid_fhtsr_dqpll] -> Bus Creator1/7  "phase_grid_fhtsr_dqpll"
  [omega_grid_fhtsr_dqpll] -> Bus Creator1/8  "omega_grid_fhtsr_dqpll"
  [omega_grid_fht_simulink_pll] -> Bus Creator1/6  "omega_grid_fht_simulink_pll"
  [phase_grid_fht_simulink_pll] -> Bus Creator1/5  "phase_grid_fht_simulink_pll"

== system pgfm_ctrl_analysis/afe_abc_inv_psm_mod2/AFE_control/afe_control/data_to_worspace_module_1/inner_current_tracking ==
  Bus Creator1 : BusCreator  Inputs=11
  m_inner_current_tracking : Outport
  wires:
  Bus Creator1/1 -> m_inner_current_tracking/1
  [isc_ref] -> Bus Creator1/7  "isc_pu_ref"
  [iz_ctrl_out] -> Bus Creator1/11  "iz_ctrl_out"
  [isb_ref] -> Bus Creator1/5  "isb_pu_ref"
  [isb] -> Bus Creator1/6  "isb_pu"
  [iz_pu_ref] -> Bus Creator1/9  "iz_pu_ref"
  [id_xi_pu] -> Bus Creator1/1  "i_xi_pu"
  [isa] -> Bus Creator1/4  "isa_pu"
  [isa_ref] -> Bus Creator1/3  "isa_pu_ref"
  [isc] -> Bus Creator1/8  "isc_pu"
  [id_eta_pu] -> Bus Creator1/2  "i_eta_pu"
  [iz_pu] -> Bus Creator1/10  "iz_pu"
